simulink model "input_response_step_ramp_quadratic"  (R2024a)
settings: Solver=VariableStepAuto  StartTime=0.0  StopTime=10.0  RelTol=1e-3
model workspace (MAT data in the model file):
  t = 1
undefined symbols (not defined in the file or in its folder): magnitude
libraries: simulink x1
settings Model: Creator=ilo_l  LastModifiedBy=ilo_l

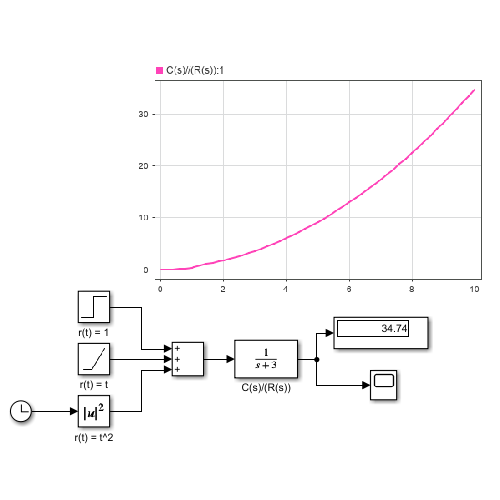
[thumbnail: Simulink's stored preview of the top-level diagram]
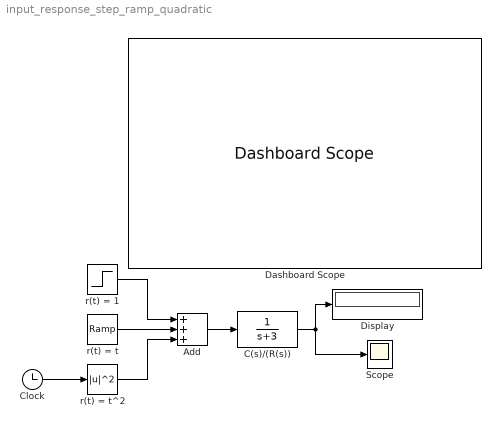
== system input_response_step_ramp_quadratic ==
  Add : Sum  Inputs=+++
  C(s)/(R(s)) : TransferFcn  Denominator=[1 3]
  Clock : Clock
  Dashboard Scope : DashboardScope  Ymax=50
  Display : Display
  Scope : Scope
  r(t) = 1 : Step  SampleTime=1
  r(t) = t : simulink/Sources/Ramp  slope=1  start=0  InitialOutput=0
  r(t) = t^2 : Math  Operator=magnitude^2
  wires:
  C(s)/(R(s))/1 -> Scope/1, Display/1
  r(t) = 1/1 -> Add/1
  r(t) = t/1 -> Add/2
  Add/1 -> C(s)/(R(s))/1
  Clock/1 -> r(t) = t^2/1
  r(t) = t^2/1 -> Add/3
